simulink model "s4_ortalama_kararlilik"  (R2023b)
settings: Solver=ode23t  StartTime=0.0  StopTime=0.11  MaxStep=1e-6  RelTol=1e-6
undefined symbols (not defined in the file): DiscIntNeverNeededParam, f_grid, K14, K34, L1_core_Rp4, L2, phase_deg4, pwm_ref_amp, pwm_ref_Ts, S4_iL1_sign, S4_int_lim, S4_Iref, S4_Iref_step, S4_Kaw, S4_Ki_c, S4_Kp_c, S4_Kr, S4_Lg_ek, S4_lp_den, S4_lp_num, S4_R_den, S4_R_num1, S4_t_step, S4_Ts_c, S4_u_lim, S6_inj_A, S6_inj_f, S6_inj_ph, Vac4_peak, Vdc4
libraries: fl_lib x11, nesl_utility x4
settings Model: Creator=burha  LastModifiedBy=burha

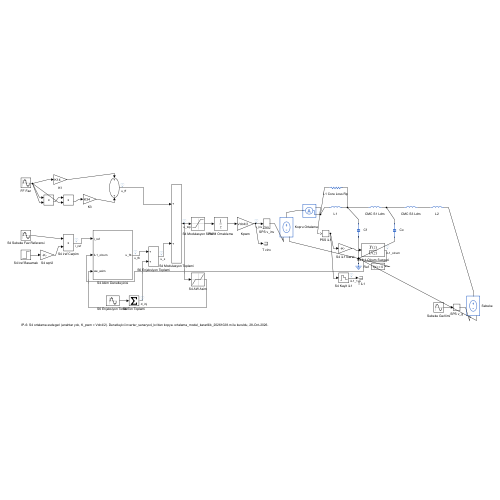
[thumbnail: Simulink's stored preview of the top-level diagram]
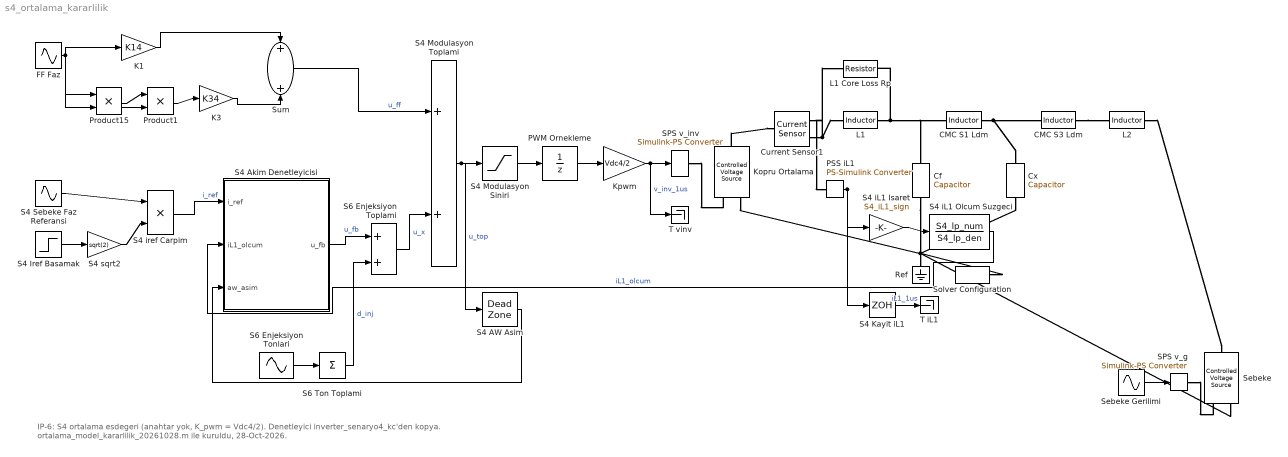
== system s4_ortalama_kararlilik ==
  note: IP-6: S4 ortalama esdegeri (anahtar yok, K_pwm = Vdc4/2). Denetleyici inverter_senaryo4_kc'den kopya. ortalama_model_kararlilik_20261028.m ile kuruldu, 28-Oct-2026.
  CMC S1 Ldm : fl_lib/Electrical/Electrical Elements/Inductor  l=EMC_Ldm_stage H  r=EMC_Rdm_stage Ohm  g=0 1/Ohm  i_specify=off  i_priority=None  i=0 A  i_nominal_specify=off  i_nominal_unit=A  i_nominal_value=1  v_specify=off  v_priority=None  v=0 V  v_nominal_specify=off  v_nominal_unit=V  v_nominal_value=1  i_L_specify=off  i_L_priority=High  i_L=0 A  i_L_nominal_specify=off  i_L_nominal_unit=A  i_L_nominal_value=1
  CMC S3 Ldm : fl_lib/Electrical/Electrical Elements/Inductor  l=EMC_Ldm_stage H  r=EMC_Rdm_stage Ohm  g=0 1/Ohm  i_specify=off  i_priority=None  i=0 A  i_nominal_specify=off  i_nominal_unit=A  i_nominal_value=1  v_specify=off  v_priority=None  v=0 V  v_nominal_specify=off  v_nominal_unit=V  v_nominal_value=1  i_L_specify=off  i_L_priority=High  i_L=0 A  i_L_nominal_specify=off  i_L_nominal_unit=A  i_L_nominal_value=1
  Cf : fl_lib/Electrical/Electrical Elements/Capacitor  c=C F  r=Cr Ohm  g=0 1/Ohm  i_specify=off  i_priority=None  i=0 A  i_nominal_specify=off  i_nominal_unit=A  i_nominal_value=1  v_specify=off  v_priority=None  v=0 V  v_nominal_specify=off  v_nominal_unit=V  v_nominal_value=1  vc_specify=off  vc_priority=High  vc=0 V  vc_nominal_specify=off  vc_nominal_unit=V  vc_nominal_value=1
  Current Sensor1 : fl_lib/Electrical/Electrical Sensors/Current Sensor
  Cx : fl_lib/Electrical/Electrical Elements/Capacitor  c=EMC_Cx_eq F  r=EMC_Rx_eq Ohm  g=0 1/Ohm  i_specify=off  i_priority=None  i=0 A  i_nominal_specify=off  i_nominal_unit=A  i_nominal_value=1  v_specify=off  v_priority=None  v=0 V  v_nominal_specify=off  v_nominal_unit=V  v_nominal_value=1  vc_specify=off  vc_priority=High  vc=0 V  vc_nominal_specify=off  vc_nominal_unit=V  vc_nominal_value=1
  FF Faz : Sin  Amplitude=pwm_ref_amp  Frequency=2*pi*f_grid  Phase=phase_deg4*pi/180  SampleTime=pwm_ref_Ts
  K1 : Gain  Gain=K14
  K3 : Gain  Gain=K34
  Kopru Ortalama : fl_lib/Electrical/Electrical Sources/Controlled Voltage Source
  Kpwm : Gain  Gain=Vdc4/2
  L1 : fl_lib/Electrical/Electrical Elements/Inductor  l=L1 H  r=L1r Ohm  g=0 1/Ohm  i_specify=off  i_priority=None  i=0 A  i_nominal_specify=off  i_nominal_unit=A  i_nominal_value=1  v_specify=off  v_priority=None  v=0 V  v_nominal_specify=off  v_nominal_unit=V  v_nominal_value=1  i_L_specify=off  i_L_priority=High  i_L=0 A  i_L_nominal_specify=off  i_L_nominal_unit=A  i_L_nominal_value=1
  L1 Core Loss Rp : fl_lib/Electrical/Electrical Elements/Resistor  R=L1_core_Rp4 Ohm  i_specify=off  i_priority=None  i=0 A  i_nominal_specify=off  i_nominal_unit=A  i_nominal_value=1  v_specify=off  v_priority=None  v=0 V  v_nominal_specify=off  v_nominal_unit=V  v_nominal_value=1
  L2 : fl_lib/Electrical/Electrical Elements/Inductor  l=L2 + S4_Lg_ek H  r=L2r Ohm  g=0 1/Ohm  i_specify=off  i_priority=None  i=0 A  i_nominal_specify=off  i_nominal_unit=A  i_nominal_value=1  v_specify=off  v_priority=None  v=0 V  v_nominal_specify=off  v_nominal_unit=V  v_nominal_value=1  i_L_specify=off  i_L_priority=High  i_L=0 A  i_L_nominal_specify=off  i_L_nominal_unit=A  i_L_nominal_value=1
  PSS iL1 : nesl_utility/PS-Simulink Converter  PhysicalDomain=network_engine_domain  SubClassName=ps_output  LeftPortType=input  RightPortType=output  PseudoPeriodic=off  Frequencies=[]  VectorFormat=inherit  Unit=A  AffineConversion=off
  PWM Ornekleme : UnitDelay  SampleTime=pwm_ref_Ts  HasFrameUpgradeWarning=on
  Product1 : Product
  Product15 : Product
  Ref : fl_lib/Electrical/Electrical Elements/Electrical Reference
  S4 AW Asim : DeadZone  LowerValue=-S4_u_lim  UpperValue=S4_u_lim
  S4 Akim Denetleyicisi : Subsystem  Description=S4 akim denetleyicisi: u_fb = Kp*e + Integrator(Ki*e - Kaw*aw) + R(z)*e. P: Ki = Kaw = Kr = 0. Dogrusallastirma (IP-6): giris i_ref / iL1_olcum, cikis u_fb.
  S4 Iref Basamak : Step  Time=S4_t_step  Before=S4_Iref  After=S4_Iref_step  SampleTime=pwm_ref_Ts
  S4 Kayit iL1 : ZeroOrderHold  SampleTime=pwm_ref_Ts
  S4 Modulasyon Siniri : Saturate  UpperLimit=S4_u_lim  LowerLimit=-S4_u_lim
  S4 Modulasyon Toplami : Sum
  S4 Sebeke Faz Referansi : Sin  Frequency=2*pi*f_grid  SampleTime=pwm_ref_Ts
  S4 iL1 Isaret : Gain  Gain=S4_iL1_sign
  S4 iL1 Olcum Suzgeci : DiscreteTransferFcn  Numerator=S4_lp_num  Denominator=S4_lp_den  SampleTime=S4_Ts_c
  S4 iref Carpim : Product
  S4 sqrt2 : Gain  Gain=sqrt(2)
  S6 Enjeksiyon Tonlari : Sin  Amplitude=S6_inj_A  Frequency=2*pi*S6_inj_f  Phase=S6_inj_ph  SampleTime=pwm_ref_Ts
  S6 Enjeksiyon Toplami : Sum
  S6 Ton Toplami : Sum  Inputs=+
  SPS v_g : nesl_utility/Simulink-PS Converter  PhysicalDomain=network_engine_domain  SubClassName=ps_input  LeftPortType=input  RightPortType=output  PseudoPeriodic=off  Frequencies=[]  NoiseDistribution=none  NoiseParameters=[]  Unit=V  AffineConversion=off  FilteringAndDerivatives=zero  SimscapeFilterOrder=1  InputFilterTimeConstant=0.001  UdotUserProvided=0
  SPS v_inv : nesl_utility/Simulink-PS Converter  PhysicalDomain=network_engine_domain  SubClassName=ps_input  LeftPortType=input  RightPortType=output  PseudoPeriodic=off  Frequencies=[]  NoiseDistribution=none  NoiseParameters=[]  Unit=V  AffineConversion=off  FilteringAndDerivatives=zero  SimscapeFilterOrder=1  InputFilterTimeConstant=0.001  UdotUserProvided=0
  Sebeke : fl_lib/Electrical/Electrical Sources/Controlled Voltage Source
  Sebeke Gerilimi : Sin  Amplitude=Vac4_peak  Frequency=2*pi*f_grid  SampleTime=0
  Solver Configuration : nesl_utility/Solver Configuration  PhysicalDomain=network_engine_domain  SubClassName=solver  LeftPortType=input  RightPortType=generic  Tones=[]  Harmonics=[]  SimulateNoise=off  Profile=off  UseLocalSampling=off  EnableSwitchedLinearOptims=on  FrequencyDomain=off  UseCCode=off  RelTol=0.001  AbsTol=0.001  MinStep=1e-09  ToWorkspace=off  RevertToSquareIcSolve=off  NumHomotopyIterations=100  PhasorMode=off  PhasorModeNumHarmonics=1  ConsistencySolver=NEWTON_XTOL_AFTER_FTOL  IndexReductionMethod=DerivativeReplacement  DoDC=off  ResidualTolerance=1e-09  ConsistencyTolSource=GLOBAL  ConsistencyAbsTol=0.001  ConsistencyRelTol=0.001  ConsistencyTolFactor=0.001  UseLocalSolver=off  LocalSolverChoice=NE_BACKWARD_EULER_ADVANCER  ResolveIndetEquations=on  FunctionEvalNumThread=1  LocalSolverSampleTime=0.001  DoFixedCost=off  MaxNonlinIter=3  MaxModeIter=2  ComputeImpulses=off  ImpulseIterations=2  LinearAlgebra=auto  LinearAlgebraNumThread=0  EquationFormulation=NE_TIME_EF  DelaysMemoryBudget=1024  AutomaticFiltering=on  FilteringTimeConstant=0.001  PartitionStorageMethod=AS_NEEDED  PartitionMemoryBudget=1024  PartitionMethod=ROBUST  MultibodyUseLocalSolver=off  MultibodyLocalSolverChoice=ODE1  MultibodyLocalSolverSampleTime=0.001
  Sum : Sum
  T iL1 : Terminator
  T vinv : Terminator
  wires:
  FF Faz/1 -> K1/1, Product15/1, Product15/2, Product1/2
  Product15/1 -> Product1/1
  Product1/1 -> K3/1
  K1/1 -> Sum/1
  K3/1 -> Sum/2
  S4 Sebeke Faz Referansi/1 -> S4 iref Carpim/1
  S4 Iref Basamak/1 -> S4 sqrt2/1
  S4 sqrt2/1 -> S4 iref Carpim/2
  S4 iref Carpim/1 -> S4 Akim Denetleyicisi/1(i_ref)  "i_ref"
  S6 Enjeksiyon Tonlari/1 -> S6 Ton Toplami/1
  S4 Akim Denetleyicisi/1(u_fb) -> S6 Enjeksiyon Toplami/1  "u_fb"
  S6 Ton Toplami/1 -> S6 Enjeksiyon Toplami/2  "d_inj"
  Sum/1 -> S4 Modulasyon Toplami/1  "u_ff"
  S6 Enjeksiyon Toplami/1 -> S4 Modulasyon Toplami/2  "u_x"
  S4 Modulasyon Toplami/1 -> S4 Modulasyon Siniri/1, S4 AW Asim/1  "u_top"
  S4 AW Asim/1 -> S4 Akim Denetleyicisi/3(aw_asim)
  S4 Modulasyon Siniri/1 -> PWM Ornekleme/1
  PWM Ornekleme/1 -> Kpwm/1
  Kpwm/1 -> SPS v_inv/1, T vinv/1  "v_inv_1us"
  Sebeke Gerilimi/1 -> SPS v_g/1
  PSS iL1/1 -> S4 iL1 Isaret/1, S4 Kayit iL1/1
  S4 iL1 Isaret/1 -> S4 iL1 Olcum Suzgeci/1
  S4 iL1 Olcum Suzgeci/1 -> S4 Akim Denetleyicisi/2(iL1_olcum)  "iL1_olcum"
  S4 Kayit iL1/1 -> T iL1/1  "iL1_1us"
  connections:
  SPS v_inv/RConn1 -- Kopru Ortalama/RConn1
  Kopru Ortalama/LConn1 -- Current Sensor1/LConn1
  L1/LConn1 -- Current Sensor1/RConn2 -- L1 Core Loss Rp/LConn1
  L1 Core Loss Rp/RConn1 -- L1/RConn1 -- Cf/LConn1 -- CMC S1 Ldm/LConn1
  Cx/LConn1 -- CMC S1 Ldm/RConn1 -- CMC S3 Ldm/LConn1
  CMC S3 Ldm/RConn1 -- L2/LConn1
  L2/RConn1 -- Sebeke/LConn1
  SPS v_g/RConn1 -- Sebeke/RConn1
  Sebeke/RConn2 -- Kopru Ortalama/RConn2 -- Cf/RConn1 -- Cx/RConn1 -- Ref/LConn1 -- Solver Configuration/RConn1
  Current Sensor1/RConn1 -- PSS iL1/LConn1

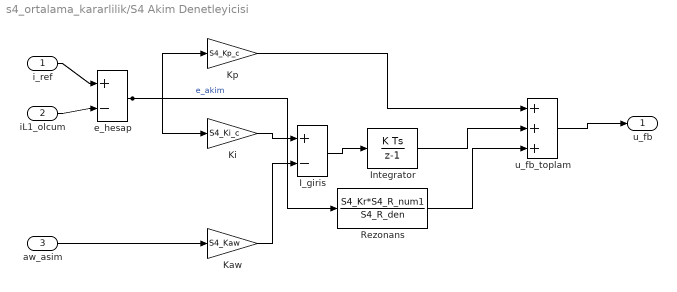
== system s4_ortalama_kararlilik/S4 Akim Denetleyicisi ==
  i_ref : Inport
  iL1_olcum : Inport  Port=2
  aw_asim : Inport  Port=3
  I_giris : Sum  Inputs=+-
  Integrator : DiscreteIntegrator  gainval=1  SampleTime=S4_Ts_c  LimitOutput=on  UpperSaturationLimit=S4_int_lim  LowerSaturationLimit=-S4_int_lim  ICPrevOutput=DiscIntNeverNeededParam  ICPrevScaledInput=DiscIntNeverNeededParam
  Kaw : Gain  Gain=S4_Kaw
  Ki : Gain  Gain=S4_Ki_c
  Kp : Gain  Gain=S4_Kp_c
  Rezonans : DiscreteTransferFcn  Numerator=S4_Kr*S4_R_num1  Denominator=S4_R_den  SampleTime=S4_Ts_c
  e_hesap : Sum  Inputs=+-
  u_fb_toplam : Sum  Inputs=+++
  u_fb : Outport
  wires:
  u_fb_toplam/1 -> u_fb/1
  Rezonans/1 -> u_fb_toplam/3
  Integrator/1 -> u_fb_toplam/2
  Kp/1 -> u_fb_toplam/1
  I_giris/1 -> Integrator/1
  Kaw/1 -> I_giris/2
  Ki/1 -> I_giris/1
  aw_asim/1 -> Kaw/1
  e_hesap/1 -> Rezonans/1, Ki/1, Kp/1  "e_akim"
  iL1_olcum/1 -> e_hesap/2
  i_ref/1 -> e_hesap/1
